simulink model "DK_V3"  (R2025b)
settings: Solver=ode23tb  StartTime=0.0  StopTime=2.0  MaxStep=1e-3  RelTol=1e-4  AbsTol=1e-6
PreLoadFcn:
  | if ~exist('P_reg','var'), P_reg=0.069500; end; if ~exist('I_reg','var'), I_reg=0.525189; end; if ~exist('D_reg','var'), D_reg=0.001681; end; if ~exist('N_reg','var'), N_reg=1000.0; end;
InitFcn:
  | if ~exist('P_reg','var'), P_reg=0.069500; end; if ~exist('I_reg','var'), I_reg=0.525189; end; if ~exist('D_reg','var'), D_reg=0.001681; end; if ~exist('N_reg','var'), N_reg=1000.0; end;
libraries: slpidlib x1
settings Model: Creator=johan  LastModifiedBy=johan

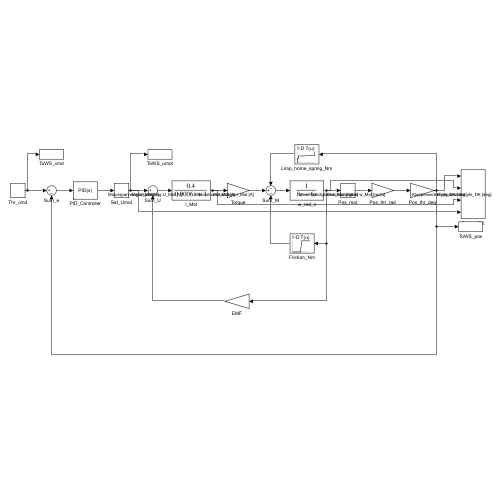
[thumbnail: Simulink's stored preview of the top-level diagram]
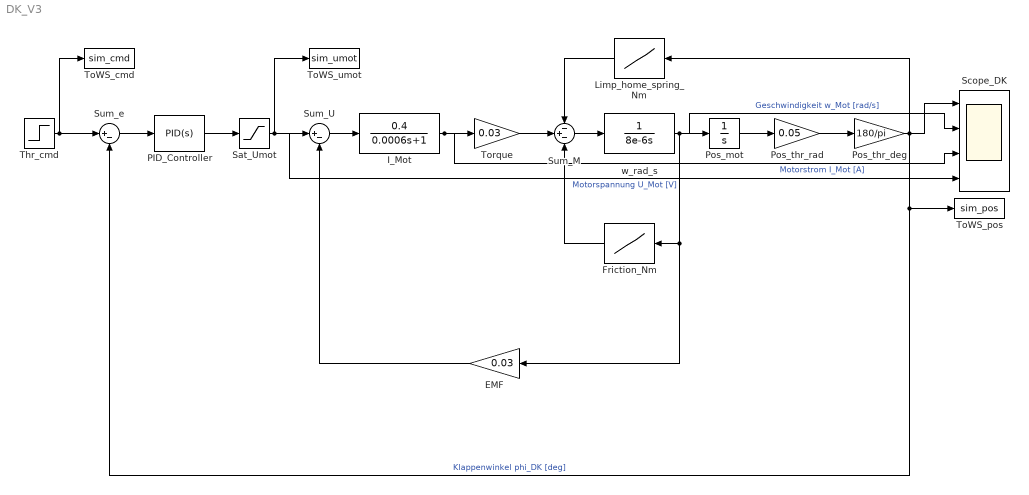
== system DK_V3 ==
  EMF : Gain  Gain=0.03
  Friction_Nm : Lookup_n-D  NumberOfTableDimensions=1  BreakpointsForDimension1=[-10, -1, 1, 10]  Table=[-0.01, -0.01, 0.01, 0.01]  InternalRulePriority=Speed  RndMeth=Simplest
  I_Mot : TransferFcn  Numerator=[0.4]  Denominator=[0.0006 1]
  Limp_home_spring_Nm : Lookup_n-D  NumberOfTableDimensions=1  BreakpointsForDimension1=[-0.1, 0, 4.9, 5.1, 90, 90.1]  Table=[-0.1, -0.0253, -0.025, 0.025, 0.029, 0.1]  InternalRulePriority=Speed  RndMeth=Simplest
  PID_Controller : slpidlib/PID Controller  Controller=PID  Form=Parallel  TimeDomain=Continuous-time  UseExternalTs=off  SampleTime=-1  IntegratorMethod=Forward Euler  FilterMethod=Forward Euler  ControllerParametersSource=internal  P=0.069500  I=0.525189  UseKiTs=off  D=0.001681  UseExternalDerivativeSource=off  N=1000.0  UseFilter=on  TunerSelectOption=Transfer Function Based (PID Tuner App)  InitialConditionSource=internal  InitialConditionForIntegrator=0  InitialConditionForFilter=0  DifferentiatorICPrevScaledInput=0  ExternalReset=none  TrackingMode=off  Kt=1  LimitOutput=off  SatLimitsSource=internal  UpperSaturationLimit=inf  LowerSaturationLimit=-inf  LinearizeAsGain=on  AntiWindupMode=none  Kb=1  LimitIntegrator=off  UpperIntegratorSaturationLimit=inf  LowerIntegratorSaturationLimit=-inf  POutMin=[]  POutMax=[]  IOutMin=[]  IOutMax=[]  DOutMin=[]  DOutMax=[]  NOutMin=[]  NOutMax=[]  SumOutMin=[]  SumOutMax=[]  SaturationOutMin=[]  SaturationOutMax=[]  PParamMin=[]  PParamMax=[]  IParamMin=[]  IParamMax=[]  DParamMin=[]  DParamMax=[]  NParamMin=[]  NParamMax=[]  KbParamMin=[]  KbParamMax=[]  KtParamMin=[]  KtParamMax=[]  KbOutMin=[]  KbOutMax=[]  KtOutMin=[]  KtOutMax=[]  IntegratorOutMin=[]  IntegratorOutMax=[]  FilterOutMin=[]  FilterOutMax=[]  SumI1OutMin=[]  SumI1OutMax=[]  SumI2OutMin=[]  SumI2OutMax=[]  SumI3OutMin=[]  SumI3OutMax=[]  SumI4OutMin=[]  SumI4OutMax=[]  SumDOutMin=[]  SumDOutMax=[]  DifferentiatorOutMin=[]  DifferentiatorOutMax=[]  FilterDiffOutCoefMin=[]  FilterDiffOutCoefMax=[]  ReciprocalOutMin=[]  ReciprocalOutMax=[]  SumDenOutMin=[]  SumDenOutMax=[]  SumNumOutMin=[]  SumNumOutMax=[]  DivideOutMin=[]  DivideOutMax=[]  UdiffTsProdOutMin=[]  UdiffTsProdOutMax=[]  NTsProdOutMin=[]  NTsProdOutMax=[]  UintegralTsProdOutMin=[]  UintegralTsProdOutMax=[]  UngainTsProdOutMin=[]  UngainTsProdOutMax=[]  ClampingZeroOutDataTypeStr=Inherit: Inherit via back propagation  ClampingZeroOutMin=[]  ClampingZeroOutMax=[]  FilterDenConstantOutDataTypeStr=Inherit: Inherit via back propagation  FilterDenConstantOutMin=[]  FilterDenConstantOutMax=[]  PCopyOutDataTypeStr=Inherit: Inherit via back propagation  PCopyOutMin=[]  PCopyOutMax=[]  NCopyOutDataTypeStr=Inherit: Inherit via back propagation  NCopyOutMin=[]  NCopyOutMax=[]  IntegratorContinuousStateAttributes=''  IntegratorStateMustResolveToSignalObject=off  IntegratorRTWStateStorageClass=Auto  FilterContinuousStateAttributes=''  FilterStateMustResolveToSignalObject=off  FilterRTWStateStorageClass=Auto  ParallelPVariant=InternalParameters  IdealPVariant=Disabled  IVariant=InternalParameters  DVariant=InternalParameters  IntegratorVariant=Continuous  SatVariant=Disabled  AWVariant=Passthrough  PCopyVariant=Disabled  TRVariant=Disabled  FdbkBlocksVariant=Forward  IdealPFdbkVariant=Disabled  SatFdbkVariant=Disabled  DerivativeFilterVariant=ContFilter  NVariant=InternalParameters  NCopyVariant=Disabled  FilterICVariant=InternalICsFilter  IntegratorICVariant=InternalICs  ExternalResetVariant=Disabled  TRSumVariant=Passthrough  SumFdbkVariant=Disabled  SumVariant=Sum_PID  TsampFilterVariant=InternalTs  TsampNgainVariant=Passthrough  TsampIntegralVariant=Disabled_SignalSpec  ExternalSaturationOutDataTypeStr=Inherit: Same as second input  DerivativeSourceVariant=ErrorSignal  PreIntVariant=InternalPreInt
  Pos_mot : Integrator  InitialCondition=10 * (pi/180) / 0.05
  Pos_thr_deg : Gain  Gain=180/pi
  Pos_thr_rad : Gain  Gain=0.05
  Sat_Umot : Saturate  UpperLimit=12  LowerLimit=-12
  Scope_DK : Scope  NumInputPorts=4
  Sum_M : Sum  Inputs=-+-
  Sum_U : Sum  Inputs=|+-
  Sum_e : Sum  Inputs=|+-
  Thr_cmd : Step  Time=0.1  Before=10  After=60  SampleTime=0
  ToWS_cmd : ToWorkspace  VariableName=sim_cmd  SampleTime=-1
  ToWS_pos : ToWorkspace  VariableName=sim_pos  SampleTime=-1
  ToWS_umot : ToWorkspace  VariableName=sim_umot  SampleTime=-1
  Torque : Gain  Gain=0.03
  w_rad_s : TransferFcn  Denominator=[8e-6 0]
  wires:
  Thr_cmd/1 -> Sum_e/1, ToWS_cmd/1
  Sum_e/1 -> PID_Controller/1
  PID_Controller/1 -> Sat_Umot/1
  Sat_Umot/1 -> Sum_U/1, ToWS_umot/1, Scope_DK/4  "Motorspannung U_Mot [V]"
  Sum_U/1 -> I_Mot/1
  I_Mot/1 -> Torque/1, Scope_DK/3  "Motorstrom I_Mot [A]"
  Torque/1 -> Sum_M/2
  Sum_M/1 -> w_rad_s/1
  w_rad_s/1 -> Friction_Nm/1, EMF/1, Pos_mot/1, Scope_DK/2  "Geschwindigkeit w_Mot [rad/s]"
  Pos_mot/1 -> Pos_thr_rad/1
  Pos_thr_rad/1 -> Pos_thr_deg/1
  Pos_thr_deg/1 -> Sum_e/2, ToWS_pos/1, Limp_home_spring_Nm/1, Scope_DK/1  "Klappenwinkel phi_DK [deg]"
  Limp_home_spring_Nm/1 -> Sum_M/1
  Friction_Nm/1 -> Sum_M/3
  EMF/1 -> Sum_U/2
